simulink model "acc_mpc"  (R2021b)
settings: Solver=ode5  StartTime=0.0  StopTime=80  FixedStep=1/20  RelTol=1e-3
PreLoadFcn:
  | mbxruntime.callbacks.PreLoadFcn(bdroot);
PostLoadFcn:
  | mbxruntime.callbacks.PostLoadFcn(bdroot);
InitFcn:
  | mbxruntime.callbacks.InitFcn(bdroot);
StartFcn:
  | mbxruntime.callbacks.StartFcn(bdroot);
StopFcn:
  | mbxruntime.callbacks.StopFcn(bdroot);
model workspace: external: MAT-File .\kea_demo_0218_cs_hws.mat (data not in the file)
undefined symbols (not defined in the file): DiscIntNeverNeededParam, kea_demo_0218_cs_1d5c9b61e8e009e5, kea_demo_0218_cs_4669f259e7287783, kea_demo_0218_cs_87ee11d7829c0052, kea_demo_0218_cs_Audi_A3_1_Dynamics_Simple_initialPitch, kea_demo_0218_cs_Audi_A3_1_Dynamics_Simple_initialRoll, kea_demo_0218_cs_Audi_A3_1_Dynamics_Simple_initialX, kea_demo_0218_cs_Audi_A3_1_Dynamics_Simple_initialY, kea_demo_0218_cs_Audi_A3_1_Dynamics_Simple_initialYaw, kea_demo_0218_cs_Audi_A3_1_Dynamics_Simple_initialZ, kea_demo_0218_cs_Audi_A3_1_PathFollower_Preview_1_PathUniqueID, kea_demo_0218_cs_Roewe_550_S_Sedan_1_Dynamics_Simple_initialX, kea_demo_0218_cs_Roewe_550_S_Sedan_1_Dynamics_Simple_initialY, kea_demo_0218_cs_Roewe_550_S_Sedan_1_Dynamics_Simple_initialYaw, kea_demo_0218_cs_Roewe_550_S_Sedan_1_Dynamics_Simple_initialZ, mbxruntime, warningInitialVelocity, x0
libraries: simulink x56, simulink_extras x18, mpcadaslib x1
(part 8 of 8)

== matlab function acc_mpc/Roewe_550_S_Sedan_1/PathFollower_Preview_1/LateralController/Calculate delta wheel/eml_delta_steering_error ==
  data: v_x_vehicle input; v_x_vehicle_Min input; t_Preview_LatCtrl input; delta_steeringwheeltotal output; v_y_vehicle input; yawrate_vehicle input; CorneringStiffness_Tyres_Front input; CorneringStiffness_Tyres_Rear input; m_vehicle_total input; inertia_z_vehicle_total input; e_Lat input size=10; Pos_x_CoG_Vehicle input; wheelbase input; RefreshCounter parameter
function delta_steeringwheeltotal = eml_delta_steering_error(v_x_vehicle,v_x_vehicle_Min,t_Preview_LatCtrl,v_y_vehicle,yawrate_vehicle,CorneringStiffness_Tyres_Front,CorneringStiffness_Tyres_Rear,m_vehicle_total,inertia_z_vehicle_total,e_Lat,Pos_x_CoG_Vehicle,wheelbase,RefreshCounter)

delta_steeringwheeltotal = emlfcn_delta_steering_error(v_x_vehicle,v_x_vehicle_Min,t_Preview_LatCtrl,v_y_vehicle,yawrate_vehicle,CorneringStiffness_Tyres_Front,CorneringStiffness_Tyres_Rear,m_vehicle_total,inertia_z_vehicle_total,e_Lat,Pos_x_CoG_Vehicle,wheelbase,RefreshCounter);

% end function

== matlab function acc_mpc/Roewe_550_S_Sedan_1/MATLAB Function ==
  data: x input; y output

    function y = calculateY(x)
    if x > 50
        y = 5;
    elseif x > 30
        y = 10;
    elseif x > 10
        y = 14;
    else
        y = 20;
    end
end

== matlab function acc_mpc/Audi_A3_1/PathFollower_Preview_1/LateralController/Calculate delta wheel/eml_delta_steering_error ==
  data: v_x_vehicle input; v_x_vehicle_Min input; t_Preview_LatCtrl input; delta_steeringwheeltotal output; v_y_vehicle input; yawrate_vehicle input; CorneringStiffness_Tyres_Front input; CorneringStiffness_Tyres_Rear input; m_vehicle_total input; inertia_z_vehicle_total input; e_Lat input size=10; Pos_x_CoG_Vehicle input; wheelbase input; RefreshCounter parameter
function delta_steeringwheeltotal = eml_delta_steering_error(v_x_vehicle,v_x_vehicle_Min,t_Preview_LatCtrl,v_y_vehicle,yawrate_vehicle,CorneringStiffness_Tyres_Front,CorneringStiffness_Tyres_Rear,m_vehicle_total,inertia_z_vehicle_total,e_Lat,Pos_x_CoG_Vehicle,wheelbase,RefreshCounter)

delta_steeringwheeltotal = emlfcn_delta_steering_error(v_x_vehicle,v_x_vehicle_Min,t_Preview_LatCtrl,v_y_vehicle,yawrate_vehicle,CorneringStiffness_Tyres_Front,CorneringStiffness_Tyres_Rear,m_vehicle_total,inertia_z_vehicle_total,e_Lat,Pos_x_CoG_Vehicle,wheelbase,RefreshCounter);

% end function
